simulink model "ASM_Traffic_MultiCore"  (R2026a)
settings: Solver=ode1  StartTime=SIM.tstart.v  StopTime=SIM.tend.v  FixedStep=SIM.StepSize.v
PostLoadFcn:
  | if any(exist('dsrtsu_mdlpostloadfcn', 'file') ~= 0), dsrtsu_mdlpostloadfcn('Execute', bdroot); end
  | try, asm_mdl_postloadfcn(bdroot, 'UpdateModel', 3600); catch, disp(lasterr); end,
InitFcn:
  | , if any(exist('rtifpga_mdlclblib', 'file') ~= 0), rtifpga_mdlclblib('Init', bdroot); end,
  | , if any(exist('dsmpb_private', 'file') ~= 0), dsmpb_private('dsmpb_mdlclblib', 'Init', bdroot); end,
model workspace (MAT data in the model file):
  asmReferencePath = [0 0.01 0.02 0.03 0.04 0.05 0.06 0.07 0.08 0.09 0.1 0.11 ... (350007 elements, 50001x7)]
  roadBounds : Simulink.Parameter (value not decoded)
  safetyAxes : Simulink.Parameter (value not decoded)
undefined symbols (not defined in the file): _to_, a0b2, ASM_BrakeHydraulics_DemoSystems, ASM_VehicleDynamics_DemoSystems, b98103fe8ad365046cd0, BrakeCircuit, controllerConfig, CPT, Crankshaft, DiscIntNeverNeededParam, dsmsi, FinalDriveAssembly, MDL, ModeSignals, mu, Pos_BrakePedal_Maneuver, rad, RefSignals, roadFamilyData, roadFamilyId, s_to_rpm, SIM, SoftECU, Suspension, Tire, Transmission
libraries: ASM_Traffic_lib x135, simulink x98, ASM_Utils_lib x77, ASM_VehicleDynamics_lib x70, ASM_Environment_lib x22, dsmpblib x20, dsmsilib x15, MDLD_Utils_lib x10, ASM_BrakeHydraulics_lib x3, sl_discontinuities x2
(part 63 of 65)

== system ASM_Traffic_MultiCore/VehicleDynamics/Plant/VehicleDynamics/VehicleMovement/ASMSignalCollector/Vehicle_Movement_Info_Car/Velocities ==
  CoGAndWheelVelocities : Inport
  v_Vehicle[x;y;z][m|s] : Inport  Port=2
  w_Vehicle[x;y;z][rad|s] : Inport  Port=3
  q_Wheel_dt[q1_Front;q2_Front;q1_Rear;q2_Rear][] : Inport  Port=4
  Bus Creator : BusCreator  Inputs=3
  Bus Selector : BusSelector  OutputSignals=v_Abs_Vehicle_CoG[x;y;z][km|h],w_CoG_VehicleBody[x;y;z][rad|s],WheelBodyVelocity,WheelBodyAngularVelocity,WheelAngularVelocity
  BusCreator1 : BusCreator  Inputs=2
  BusCreator2 : BusCreator  Inputs=2
  BusCreator4 : BusCreator  Inputs=3
  BusCreator5 : BusCreator  Inputs=1
  BusCreator6 : BusCreator  Inputs=1
  BusCreator7 : BusCreator  Inputs=2
  BusCreator8 : BusCreator  Inputs=3
  Selector : Selector  InputPortWidth=3  IndexOptions=Index vector (dialog)  Indices=[1 2]  OutputSizes=1
      settings: AttributesFormatString=Elements: %<Elements>
  VectorLabel : Subsystem
  VectorLabel3 : Subsystem
  VectorLabel4 : Subsystem
  "[m|s]_to_[km|h]" : Gain  Gain=3.6
  "[rad]_to_[deg]" : Gain  Gain=180/pi
  "[rad]_to_[deg]1" : Gain  Gain=180/pi
  v_Vehicle_and_AngleSideSlip : Subsystem
  Velocities : Outport  VectorParamsAs1DForOutWhenUnconnected=off
  wires:
  VectorLabel4/1(out) -> BusCreator8/3
  q_Wheel_dt[q1_Front;q2_Front;q1_Rear;q2_Rear][]/1 -> VectorLabel4/1(in)
  "[rad]_to_[deg]1"/1 -> BusCreator8/2  "w_Vehicle[x;y;z][deg|s]"
  "[rad]_to_[deg]"/1 -> VectorLabel3/1(in)
  w_Vehicle[x;y;z][rad|s]/1 -> "[rad]_to_[deg]1"/1
  BusCreator8/1 -> Bus Creator/3  "Generalized"
  v_Vehicle[x;y;z][m|s]/1 -> "[m|s]_to_[km|h]"/1
  "[m|s]_to_[km|h]"/1 -> BusCreator8/1  "v_Vehicle[x;y;z][km|h]"
  CoGAndWheelVelocities/1 -> Bus Selector/1
  BusCreator2/1 -> Bus Creator/1  "Vehicle"
  BusCreator4/1 -> BusCreator2/1  "Linear"
  BusCreator5/1 -> BusCreator2/2  "Angular"
  VectorLabel3/1(out) -> BusCreator5/1
  Bus Creator/1 -> Velocities/1  "Velocities"
  BusCreator1/1 -> Bus Creator/2  "Wheels"
  BusCreator7/1 -> BusCreator1/2  "Angular"
  Bus Selector/1 -> VectorLabel/1(in), Selector/1  "<v_Abs_Vehicle_CoG[x;y;z][km|h]>"
  BusCreator6/1 -> BusCreator1/1  "Linear"
  v_Vehicle_and_AngleSideSlip/1(v_Vehicle[km|h]) -> BusCreator4/2  "v_Total_Vehicle[km|h]"
  VectorLabel/1(out) -> BusCreator4/1
  Bus Selector/2 -> "[rad]_to_[deg]"/1  "<w_CoG_VehicleBody[x;y;z][rad|s]>"
  Bus Selector/3 -> BusCreator6/1  "<WheelBodyVelocity>"
  Bus Selector/4 -> BusCreator7/1  "<WheelBodyAngularVelocity>"
  Bus Selector/5 -> BusCreator7/2  "<WheelAngularVelocity>"
  Selector/1 -> v_Vehicle_and_AngleSideSlip/1(v_Vehicle[x;y][km|h])
  v_Vehicle_and_AngleSideSlip/2(Angle_SideSlip_Vehicle[deg]) -> BusCreator4/3  "Angle_SideSlip_Vehicle[deg]"

== system ASM_Traffic_MultiCore/DomainControl/DriverAssistance/Control/SoftECU_ACC/Soft_ECU_ACC/Map_Inputs/Maneuver/pos_edge_detection ==
  In1 : Inport
  Memory : Memory
  Relational Operator : RelationalOperator  Operator=>  OutDataTypeStr=boolean  InputSameDT=off
  Out1 : Outport  VectorParamsAs1DForOutWhenUnconnected=off
  wires:
  In1/1 -> Relational Operator/1, Memory/1
  Relational Operator/1 -> Out1/1
  Memory/1 -> Relational Operator/2

== system ASM_Traffic_MultiCore/DomainControl/DriverAssistance/Control/SoftECU_ACC/Soft_ECU_ACC/Map_Inputs/Maneuver/pos_edge_detection1 ==
  In1 : Inport
  Memory : Memory
  Relational Operator : RelationalOperator  Operator=>  OutDataTypeStr=boolean  InputSameDT=off
  Out1 : Outport  VectorParamsAs1DForOutWhenUnconnected=off
  wires:
  Memory/1 -> Relational Operator/2
  Relational Operator/1 -> Out1/1
  In1/1 -> Memory/1, Relational Operator/1

== system ASM_Traffic_MultiCore/DomainControl/DriverAssistance/Control/SoftECU_ACC/Soft_ECU_ACC/Map_Inputs/Maneuver/pos_edge_detection2 ==
  In1 : Inport
  Memory : Memory
  Relational Operator : RelationalOperator  Operator=>  OutDataTypeStr=boolean  InputSameDT=off
  Out1 : Outport  VectorParamsAs1DForOutWhenUnconnected=off
  wires:
  In1/1 -> Relational Operator/1, Memory/1
  Relational Operator/1 -> Out1/1
  Memory/1 -> Relational Operator/2

== system ASM_Traffic_MultiCore/DomainControl/DriverAssistance/Control/SoftECU_ACC/Soft_ECU_ACC/Map_Inputs/Maneuver/pos_edge_detection3 ==
  In1 : Inport
  Memory : Memory
  Relational Operator : RelationalOperator  Operator=>  OutDataTypeStr=boolean  InputSameDT=off
  Out1 : Outport  VectorParamsAs1DForOutWhenUnconnected=off
  wires:
  Memory/1 -> Relational Operator/2
  Relational Operator/1 -> Out1/1
  In1/1 -> Memory/1, Relational Operator/1

== system ASM_Traffic_MultiCore/Environment/GroundTruth/UserInterface/PAR_Plant/Fellow_Vehicles/Lightstates_Fellow1/Indicator_State[]/ASM_OSI_Mapping ==
  Fellow_TurnLights[] : Inport
  Table_ASM_To_OSI : Lookup_n-D  NumberOfTableDimensions=1  BreakpointsForDimension1=[0,1,2,3]  Table=[2,3,4,5]  InterpMethod=Nearest  InternalRulePriority=Speed  RndMeth=Simplest
  Indicator_State[] : Outport  VectorParamsAs1DForOutWhenUnconnected=off
  wires:
  Table_ASM_To_OSI/1 -> Indicator_State[]/1
  Fellow_TurnLights[]/1 -> Table_ASM_To_OSI/1

== system ASM_Traffic_MultiCore/Environment/GroundTruth/UserInterface/PAR_Plant/Fellow_Vehicles/Lightstates_Fellow10/Indicator_State[]/ASM_OSI_Mapping ==
  Fellow_TurnLights[] : Inport
  Table_ASM_To_OSI : Lookup_n-D  NumberOfTableDimensions=1  BreakpointsForDimension1=[0,1,2,3]  Table=[2,3,4,5]  InterpMethod=Nearest  InternalRulePriority=Speed  RndMeth=Simplest
  Indicator_State[] : Outport  VectorParamsAs1DForOutWhenUnconnected=off
  wires:
  Fellow_TurnLights[]/1 -> Table_ASM_To_OSI/1
  Table_ASM_To_OSI/1 -> Indicator_State[]/1

== system ASM_Traffic_MultiCore/Environment/GroundTruth/UserInterface/PAR_Plant/Fellow_Vehicles/Lightstates_Fellow11/Indicator_State[]/ASM_OSI_Mapping ==
  Fellow_TurnLights[] : Inport
  Table_ASM_To_OSI : Lookup_n-D  NumberOfTableDimensions=1  BreakpointsForDimension1=[0,1,2,3]  Table=[2,3,4,5]  InterpMethod=Nearest  InternalRulePriority=Speed  RndMeth=Simplest
  Indicator_State[] : Outport  VectorParamsAs1DForOutWhenUnconnected=off
  wires:
  Table_ASM_To_OSI/1 -> Indicator_State[]/1
  Fellow_TurnLights[]/1 -> Table_ASM_To_OSI/1

== system ASM_Traffic_MultiCore/Environment/GroundTruth/UserInterface/PAR_Plant/Fellow_Vehicles/Lightstates_Fellow12/Indicator_State[]/ASM_OSI_Mapping ==
  Fellow_TurnLights[] : Inport
  Table_ASM_To_OSI : Lookup_n-D  NumberOfTableDimensions=1  BreakpointsForDimension1=[0,1,2,3]  Table=[2,3,4,5]  InterpMethod=Nearest  InternalRulePriority=Speed  RndMeth=Simplest
  Indicator_State[] : Outport  VectorParamsAs1DForOutWhenUnconnected=off
  wires:
  Fellow_TurnLights[]/1 -> Table_ASM_To_OSI/1
  Table_ASM_To_OSI/1 -> Indicator_State[]/1

== system ASM_Traffic_MultiCore/Environment/GroundTruth/UserInterface/PAR_Plant/Fellow_Vehicles/Lightstates_Fellow13/Indicator_State[]/ASM_OSI_Mapping ==
  Fellow_TurnLights[] : Inport
  Table_ASM_To_OSI : Lookup_n-D  NumberOfTableDimensions=1  BreakpointsForDimension1=[0,1,2,3]  Table=[2,3,4,5]  InterpMethod=Nearest  InternalRulePriority=Speed  RndMeth=Simplest
  Indicator_State[] : Outport  VectorParamsAs1DForOutWhenUnconnected=off
  wires:
  Table_ASM_To_OSI/1 -> Indicator_State[]/1
  Fellow_TurnLights[]/1 -> Table_ASM_To_OSI/1

== system ASM_Traffic_MultiCore/Environment/GroundTruth/UserInterface/PAR_Plant/Fellow_Vehicles/Lightstates_Fellow14/Indicator_State[]/ASM_OSI_Mapping ==
  Fellow_TurnLights[] : Inport
  Table_ASM_To_OSI : Lookup_n-D  NumberOfTableDimensions=1  BreakpointsForDimension1=[0,1,2,3]  Table=[2,3,4,5]  InterpMethod=Nearest  InternalRulePriority=Speed  RndMeth=Simplest
  Indicator_State[] : Outport  VectorParamsAs1DForOutWhenUnconnected=off
  wires:
  Fellow_TurnLights[]/1 -> Table_ASM_To_OSI/1
  Table_ASM_To_OSI/1 -> Indicator_State[]/1

== system ASM_Traffic_MultiCore/Environment/GroundTruth/UserInterface/PAR_Plant/Fellow_Vehicles/Lightstates_Fellow15/Indicator_State[]/ASM_OSI_Mapping ==
  Fellow_TurnLights[] : Inport
  Table_ASM_To_OSI : Lookup_n-D  NumberOfTableDimensions=1  BreakpointsForDimension1=[0,1,2,3]  Table=[2,3,4,5]  InterpMethod=Nearest  InternalRulePriority=Speed  RndMeth=Simplest
  Indicator_State[] : Outport  VectorParamsAs1DForOutWhenUnconnected=off
  wires:
  Table_ASM_To_OSI/1 -> Indicator_State[]/1
  Fellow_TurnLights[]/1 -> Table_ASM_To_OSI/1

== system ASM_Traffic_MultiCore/Environment/GroundTruth/UserInterface/PAR_Plant/Fellow_Vehicles/Lightstates_Fellow16/Indicator_State[]/ASM_OSI_Mapping ==
  Fellow_TurnLights[] : Inport
  Table_ASM_To_OSI : Lookup_n-D  NumberOfTableDimensions=1  BreakpointsForDimension1=[0,1,2,3]  Table=[2,3,4,5]  InterpMethod=Nearest  InternalRulePriority=Speed  RndMeth=Simplest
  Indicator_State[] : Outport  VectorParamsAs1DForOutWhenUnconnected=off
  wires:
  Fellow_TurnLights[]/1 -> Table_ASM_To_OSI/1
  Table_ASM_To_OSI/1 -> Indicator_State[]/1

== system ASM_Traffic_MultiCore/Environment/GroundTruth/UserInterface/PAR_Plant/Fellow_Vehicles/Lightstates_Fellow17/Indicator_State[]/ASM_OSI_Mapping ==
  Fellow_TurnLights[] : Inport
  Table_ASM_To_OSI : Lookup_n-D  NumberOfTableDimensions=1  BreakpointsForDimension1=[0,1,2,3]  Table=[2,3,4,5]  InterpMethod=Nearest  InternalRulePriority=Speed  RndMeth=Simplest
  Indicator_State[] : Outport  VectorParamsAs1DForOutWhenUnconnected=off
  wires:
  Table_ASM_To_OSI/1 -> Indicator_State[]/1
  Fellow_TurnLights[]/1 -> Table_ASM_To_OSI/1

== system ASM_Traffic_MultiCore/Environment/GroundTruth/UserInterface/PAR_Plant/Fellow_Vehicles/Lightstates_Fellow18/Indicator_State[]/ASM_OSI_Mapping ==
  Fellow_TurnLights[] : Inport
  Table_ASM_To_OSI : Lookup_n-D  NumberOfTableDimensions=1  BreakpointsForDimension1=[0,1,2,3]  Table=[2,3,4,5]  InterpMethod=Nearest  InternalRulePriority=Speed  RndMeth=Simplest
  Indicator_State[] : Outport  VectorParamsAs1DForOutWhenUnconnected=off
  wires:
  Fellow_TurnLights[]/1 -> Table_ASM_To_OSI/1
  Table_ASM_To_OSI/1 -> Indicator_State[]/1

== system ASM_Traffic_MultiCore/Environment/GroundTruth/UserInterface/PAR_Plant/Fellow_Vehicles/Lightstates_Fellow19/Indicator_State[]/ASM_OSI_Mapping ==
  Fellow_TurnLights[] : Inport
  Table_ASM_To_OSI : Lookup_n-D  NumberOfTableDimensions=1  BreakpointsForDimension1=[0,1,2,3]  Table=[2,3,4,5]  InterpMethod=Nearest  InternalRulePriority=Speed  RndMeth=Simplest
  Indicator_State[] : Outport  VectorParamsAs1DForOutWhenUnconnected=off
  wires:
  Table_ASM_To_OSI/1 -> Indicator_State[]/1
  Fellow_TurnLights[]/1 -> Table_ASM_To_OSI/1

== system ASM_Traffic_MultiCore/Environment/GroundTruth/UserInterface/PAR_Plant/Fellow_Vehicles/Lightstates_Fellow2/Indicator_State[]/ASM_OSI_Mapping ==
  Fellow_TurnLights[] : Inport
  Table_ASM_To_OSI : Lookup_n-D  NumberOfTableDimensions=1  BreakpointsForDimension1=[0,1,2,3]  Table=[2,3,4,5]  InterpMethod=Nearest  InternalRulePriority=Speed  RndMeth=Simplest
  Indicator_State[] : Outport  VectorParamsAs1DForOutWhenUnconnected=off
  wires:
  Fellow_TurnLights[]/1 -> Table_ASM_To_OSI/1
  Table_ASM_To_OSI/1 -> Indicator_State[]/1

== system ASM_Traffic_MultiCore/Environment/GroundTruth/UserInterface/PAR_Plant/Fellow_Vehicles/Lightstates_Fellow20/Indicator_State[]/ASM_OSI_Mapping ==
  Fellow_TurnLights[] : Inport
  Table_ASM_To_OSI : Lookup_n-D  NumberOfTableDimensions=1  BreakpointsForDimension1=[0,1,2,3]  Table=[2,3,4,5]  InterpMethod=Nearest  InternalRulePriority=Speed  RndMeth=Simplest
  Indicator_State[] : Outport  VectorParamsAs1DForOutWhenUnconnected=off
  wires:
  Fellow_TurnLights[]/1 -> Table_ASM_To_OSI/1
  Table_ASM_To_OSI/1 -> Indicator_State[]/1

== system ASM_Traffic_MultiCore/Environment/GroundTruth/UserInterface/PAR_Plant/Fellow_Vehicles/Lightstates_Fellow21/Indicator_State[]/ASM_OSI_Mapping ==
  Fellow_TurnLights[] : Inport
  Table_ASM_To_OSI : Lookup_n-D  NumberOfTableDimensions=1  BreakpointsForDimension1=[0,1,2,3]  Table=[2,3,4,5]  InterpMethod=Nearest  InternalRulePriority=Speed  RndMeth=Simplest
  Indicator_State[] : Outport  VectorParamsAs1DForOutWhenUnconnected=off
  wires:
  Table_ASM_To_OSI/1 -> Indicator_State[]/1
  Fellow_TurnLights[]/1 -> Table_ASM_To_OSI/1

== system ASM_Traffic_MultiCore/Environment/GroundTruth/UserInterface/PAR_Plant/Fellow_Vehicles/Lightstates_Fellow22/Indicator_State[]/ASM_OSI_Mapping ==
  Fellow_TurnLights[] : Inport
  Table_ASM_To_OSI : Lookup_n-D  NumberOfTableDimensions=1  BreakpointsForDimension1=[0,1,2,3]  Table=[2,3,4,5]  InterpMethod=Nearest  InternalRulePriority=Speed  RndMeth=Simplest
  Indicator_State[] : Outport  VectorParamsAs1DForOutWhenUnconnected=off
  wires:
  Fellow_TurnLights[]/1 -> Table_ASM_To_OSI/1
  Table_ASM_To_OSI/1 -> Indicator_State[]/1

== system ASM_Traffic_MultiCore/Environment/GroundTruth/UserInterface/PAR_Plant/Fellow_Vehicles/Lightstates_Fellow23/Indicator_State[]/ASM_OSI_Mapping ==
  Fellow_TurnLights[] : Inport
  Table_ASM_To_OSI : Lookup_n-D  NumberOfTableDimensions=1  BreakpointsForDimension1=[0,1,2,3]  Table=[2,3,4,5]  InterpMethod=Nearest  InternalRulePriority=Speed  RndMeth=Simplest
  Indicator_State[] : Outport  VectorParamsAs1DForOutWhenUnconnected=off
  wires:
  Table_ASM_To_OSI/1 -> Indicator_State[]/1
  Fellow_TurnLights[]/1 -> Table_ASM_To_OSI/1

== system ASM_Traffic_MultiCore/Environment/GroundTruth/UserInterface/PAR_Plant/Fellow_Vehicles/Lightstates_Fellow24/Indicator_State[]/ASM_OSI_Mapping ==
  Fellow_TurnLights[] : Inport
  Table_ASM_To_OSI : Lookup_n-D  NumberOfTableDimensions=1  BreakpointsForDimension1=[0,1,2,3]  Table=[2,3,4,5]  InterpMethod=Nearest  InternalRulePriority=Speed  RndMeth=Simplest
  Indicator_State[] : Outport  VectorParamsAs1DForOutWhenUnconnected=off
  wires:
  Fellow_TurnLights[]/1 -> Table_ASM_To_OSI/1
  Table_ASM_To_OSI/1 -> Indicator_State[]/1

== system ASM_Traffic_MultiCore/Environment/GroundTruth/UserInterface/PAR_Plant/Fellow_Vehicles/Lightstates_Fellow25/Indicator_State[]/ASM_OSI_Mapping ==
  Fellow_TurnLights[] : Inport
  Table_ASM_To_OSI : Lookup_n-D  NumberOfTableDimensions=1  BreakpointsForDimension1=[0,1,2,3]  Table=[2,3,4,5]  InterpMethod=Nearest  InternalRulePriority=Speed  RndMeth=Simplest
  Indicator_State[] : Outport  VectorParamsAs1DForOutWhenUnconnected=off
  wires:
  Table_ASM_To_OSI/1 -> Indicator_State[]/1
  Fellow_TurnLights[]/1 -> Table_ASM_To_OSI/1

== system ASM_Traffic_MultiCore/Environment/GroundTruth/UserInterface/PAR_Plant/Fellow_Vehicles/Lightstates_Fellow26/Indicator_State[]/ASM_OSI_Mapping ==
  Fellow_TurnLights[] : Inport
  Table_ASM_To_OSI : Lookup_n-D  NumberOfTableDimensions=1  BreakpointsForDimension1=[0,1,2,3]  Table=[2,3,4,5]  InterpMethod=Nearest  InternalRulePriority=Speed  RndMeth=Simplest
  Indicator_State[] : Outport  VectorParamsAs1DForOutWhenUnconnected=off
  wires:
  Fellow_TurnLights[]/1 -> Table_ASM_To_OSI/1
  Table_ASM_To_OSI/1 -> Indicator_State[]/1

== system ASM_Traffic_MultiCore/Environment/GroundTruth/UserInterface/PAR_Plant/Fellow_Vehicles/Lightstates_Fellow27/Indicator_State[]/ASM_OSI_Mapping ==
  Fellow_TurnLights[] : Inport
  Table_ASM_To_OSI : Lookup_n-D  NumberOfTableDimensions=1  BreakpointsForDimension1=[0,1,2,3]  Table=[2,3,4,5]  InterpMethod=Nearest  InternalRulePriority=Speed  RndMeth=Simplest
  Indicator_State[] : Outport  VectorParamsAs1DForOutWhenUnconnected=off
  wires:
  Table_ASM_To_OSI/1 -> Indicator_State[]/1
  Fellow_TurnLights[]/1 -> Table_ASM_To_OSI/1

== system ASM_Traffic_MultiCore/Environment/GroundTruth/UserInterface/PAR_Plant/Fellow_Vehicles/Lightstates_Fellow28/Indicator_State[]/ASM_OSI_Mapping ==
  Fellow_TurnLights[] : Inport
  Table_ASM_To_OSI : Lookup_n-D  NumberOfTableDimensions=1  BreakpointsForDimension1=[0,1,2,3]  Table=[2,3,4,5]  InterpMethod=Nearest  InternalRulePriority=Speed  RndMeth=Simplest
  Indicator_State[] : Outport  VectorParamsAs1DForOutWhenUnconnected=off
  wires:
  Fellow_TurnLights[]/1 -> Table_ASM_To_OSI/1
  Table_ASM_To_OSI/1 -> Indicator_State[]/1

== system ASM_Traffic_MultiCore/Environment/GroundTruth/UserInterface/PAR_Plant/Fellow_Vehicles/Lightstates_Fellow29/Indicator_State[]/ASM_OSI_Mapping ==
  Fellow_TurnLights[] : Inport
  Table_ASM_To_OSI : Lookup_n-D  NumberOfTableDimensions=1  BreakpointsForDimension1=[0,1,2,3]  Table=[2,3,4,5]  InterpMethod=Nearest  InternalRulePriority=Speed  RndMeth=Simplest
  Indicator_State[] : Outport  VectorParamsAs1DForOutWhenUnconnected=off
  wires:
  Table_ASM_To_OSI/1 -> Indicator_State[]/1
  Fellow_TurnLights[]/1 -> Table_ASM_To_OSI/1

== system ASM_Traffic_MultiCore/Environment/GroundTruth/UserInterface/PAR_Plant/Fellow_Vehicles/Lightstates_Fellow3/Indicator_State[]/ASM_OSI_Mapping ==
  Fellow_TurnLights[] : Inport
  Table_ASM_To_OSI : Lookup_n-D  NumberOfTableDimensions=1  BreakpointsForDimension1=[0,1,2,3]  Table=[2,3,4,5]  InterpMethod=Nearest  InternalRulePriority=Speed  RndMeth=Simplest
  Indicator_State[] : Outport  VectorParamsAs1DForOutWhenUnconnected=off
  wires:
  Table_ASM_To_OSI/1 -> Indicator_State[]/1
  Fellow_TurnLights[]/1 -> Table_ASM_To_OSI/1

== system ASM_Traffic_MultiCore/Environment/GroundTruth/UserInterface/PAR_Plant/Fellow_Vehicles/Lightstates_Fellow30/Indicator_State[]/ASM_OSI_Mapping ==
  Fellow_TurnLights[] : Inport
  Table_ASM_To_OSI : Lookup_n-D  NumberOfTableDimensions=1  BreakpointsForDimension1=[0,1,2,3]  Table=[2,3,4,5]  InterpMethod=Nearest  InternalRulePriority=Speed  RndMeth=Simplest
  Indicator_State[] : Outport  VectorParamsAs1DForOutWhenUnconnected=off
  wires:
  Fellow_TurnLights[]/1 -> Table_ASM_To_OSI/1
  Table_ASM_To_OSI/1 -> Indicator_State[]/1

== system ASM_Traffic_MultiCore/Environment/GroundTruth/UserInterface/PAR_Plant/Fellow_Vehicles/Lightstates_Fellow4/Indicator_State[]/ASM_OSI_Mapping ==
  Fellow_TurnLights[] : Inport
  Table_ASM_To_OSI : Lookup_n-D  NumberOfTableDimensions=1  BreakpointsForDimension1=[0,1,2,3]  Table=[2,3,4,5]  InterpMethod=Nearest  InternalRulePriority=Speed  RndMeth=Simplest
  Indicator_State[] : Outport  VectorParamsAs1DForOutWhenUnconnected=off
  wires:
  Fellow_TurnLights[]/1 -> Table_ASM_To_OSI/1
  Table_ASM_To_OSI/1 -> Indicator_State[]/1

== system ASM_Traffic_MultiCore/Environment/GroundTruth/UserInterface/PAR_Plant/Fellow_Vehicles/Lightstates_Fellow5/Indicator_State[]/ASM_OSI_Mapping ==
  Fellow_TurnLights[] : Inport
  Table_ASM_To_OSI : Lookup_n-D  NumberOfTableDimensions=1  BreakpointsForDimension1=[0,1,2,3]  Table=[2,3,4,5]  InterpMethod=Nearest  InternalRulePriority=Speed  RndMeth=Simplest
  Indicator_State[] : Outport  VectorParamsAs1DForOutWhenUnconnected=off
  wires:
  Table_ASM_To_OSI/1 -> Indicator_State[]/1
  Fellow_TurnLights[]/1 -> Table_ASM_To_OSI/1

== system ASM_Traffic_MultiCore/Environment/GroundTruth/UserInterface/PAR_Plant/Fellow_Vehicles/Lightstates_Fellow6/Indicator_State[]/ASM_OSI_Mapping ==
  Fellow_TurnLights[] : Inport
  Table_ASM_To_OSI : Lookup_n-D  NumberOfTableDimensions=1  BreakpointsForDimension1=[0,1,2,3]  Table=[2,3,4,5]  InterpMethod=Nearest  InternalRulePriority=Speed  RndMeth=Simplest
  Indicator_State[] : Outport  VectorParamsAs1DForOutWhenUnconnected=off
  wires:
  Fellow_TurnLights[]/1 -> Table_ASM_To_OSI/1
  Table_ASM_To_OSI/1 -> Indicator_State[]/1

== system ASM_Traffic_MultiCore/Environment/GroundTruth/UserInterface/PAR_Plant/Fellow_Vehicles/Lightstates_Fellow7/Indicator_State[]/ASM_OSI_Mapping ==
  Fellow_TurnLights[] : Inport
  Table_ASM_To_OSI : Lookup_n-D  NumberOfTableDimensions=1  BreakpointsForDimension1=[0,1,2,3]  Table=[2,3,4,5]  InterpMethod=Nearest  InternalRulePriority=Speed  RndMeth=Simplest
  Indicator_State[] : Outport  VectorParamsAs1DForOutWhenUnconnected=off
  wires:
  Table_ASM_To_OSI/1 -> Indicator_State[]/1
  Fellow_TurnLights[]/1 -> Table_ASM_To_OSI/1

== system ASM_Traffic_MultiCore/Environment/GroundTruth/UserInterface/PAR_Plant/Fellow_Vehicles/Lightstates_Fellow8/Indicator_State[]/ASM_OSI_Mapping ==
  Fellow_TurnLights[] : Inport
  Table_ASM_To_OSI : Lookup_n-D  NumberOfTableDimensions=1  BreakpointsForDimension1=[0,1,2,3]  Table=[2,3,4,5]  InterpMethod=Nearest  InternalRulePriority=Speed  RndMeth=Simplest
  Indicator_State[] : Outport  VectorParamsAs1DForOutWhenUnconnected=off
  wires:
  Fellow_TurnLights[]/1 -> Table_ASM_To_OSI/1
  Table_ASM_To_OSI/1 -> Indicator_State[]/1

== system ASM_Traffic_MultiCore/Environment/GroundTruth/UserInterface/PAR_Plant/Fellow_Vehicles/Lightstates_Fellow9/Indicator_State[]/ASM_OSI_Mapping ==
  Fellow_TurnLights[] : Inport
  Table_ASM_To_OSI : Lookup_n-D  NumberOfTableDimensions=1  BreakpointsForDimension1=[0,1,2,3]  Table=[2,3,4,5]  InterpMethod=Nearest  InternalRulePriority=Speed  RndMeth=Simplest
  Indicator_State[] : Outport  VectorParamsAs1DForOutWhenUnconnected=off
  wires:
  Table_ASM_To_OSI/1 -> Indicator_State[]/1
  Fellow_TurnLights[]/1 -> Table_ASM_To_OSI/1

== system ASM_Traffic_MultiCore/Environment/Sensors/PlantModel/Object_Sensor_2D/ObjectData/Sensor1/Object_Custom_Values/Vectorize_Signals ==
  SensorOutput1 : Inport
  SensorOutput2 : Inport  Port=2
  SensorOutput3 : Inport  Port=3
  Bus Creator : BusCreator  Inputs=2
  Bus Selector : BusSelector  OutputSignals=SensorOutput.Object1.Object_Valid[0|1],SensorOutput.Object2.Object_Valid[0|1],SensorOutput.Object3.Object_Valid[0|1],SensorOutput.Object4.Object_Valid[0|1],SensorOutput.Object5.Object_Valid[0|1]
  Bus Selector1 : BusSelector  OutputSignals=SensorOutput.Object1.Object_Valid[0|1],SensorOutput.Object2.Object_Valid[0|1],SensorOutput.Object3.Object_Valid[0|1],SensorOutput.Object4.Object_Valid[0|1],SensorOutput.Object5.Object_Valid[0|1]
  Bus Selector2 : BusSelector  OutputSignals=SensorOutput.Object1.Object_Valid[0|1],SensorOutput.Object2.Object_Valid[0|1],SensorOutput.Object3.Object_Valid[0|1],SensorOutput.Object4.Object_Valid[0|1],SensorOutput.Object5.Object_Valid[0|1]
  Bus Selector3 : BusSelector  OutputSignals=SensorOutput.Object1.CustomValues[],SensorOutput.Object2.CustomValues[],SensorOutput.Object3.CustomValues[],SensorOutput.Object4.CustomValues[],SensorOutput.Object5.CustomValues[]
  Bus Selector4 : BusSelector  OutputSignals=SensorOutput.Object1.CustomValues[],SensorOutput.Object2.CustomValues[],SensorOutput.Object3.CustomValues[],SensorOutput.Object4.CustomValues[],SensorOutput.Object5.CustomValues[]
  Bus Selector5 : BusSelector  OutputSignals=SensorOutput.Object1.CustomValues[],SensorOutput.Object2.CustomValues[],SensorOutput.Object3.CustomValues[],SensorOutput.Object4.CustomValues[],SensorOutput.Object5.CustomValues[]
  Mux : Mux  Inputs=15
  Mux1 : Mux  Inputs=15
  Vectorized_Custom_Values : Outport  VectorParamsAs1DForOutWhenUnconnected=off
  wires:
  Bus Creator/1 -> Vectorized_Custom_Values/1
  Bus Selector5/5 -> Mux1/15  "<CustomValues[]>"
  Bus Selector5/4 -> Mux1/14  "<CustomValues[]>"
  Bus Selector5/3 -> Mux1/13  "<CustomValues[]>"
  Bus Selector5/2 -> Mux1/12  "<CustomValues[]>"
  Bus Selector5/1 -> Mux1/11  "<CustomValues[]>"
  Bus Selector4/5 -> Mux1/10  "<CustomValues[]>"
  Bus Selector4/4 -> Mux1/9  "<CustomValues[]>"
  Bus Selector4/3 -> Mux1/8  "<CustomValues[]>"
  Bus Selector4/2 -> Mux1/7  "<CustomValues[]>"
  Bus Selector4/1 -> Mux1/6  "<CustomValues[]>"
  Bus Selector3/5 -> Mux1/5  "<CustomValues[]>"
  Bus Selector3/4 -> Mux1/4  "<CustomValues[]>"
  Bus Selector3/3 -> Mux1/3  "<CustomValues[]>"
  Bus Selector3/2 -> Mux1/2  "<CustomValues[]>"
  Bus Selector3/1 -> Mux1/1  "<CustomValues[]>"
  Bus Selector2/5 -> Mux/15  "<Object_Valid[0|1]>"
  Bus Selector2/4 -> Mux/14  "<Object_Valid[0|1]>"
  Bus Selector2/3 -> Mux/13  "<Object_Valid[0|1]>"
  Bus Selector2/2 -> Mux/12  "<Object_Valid[0|1]>"
  Bus Selector2/1 -> Mux/11  "<Object_Valid[0|1]>"
  Bus Selector1/5 -> Mux/10  "<Object_Valid[0|1]>"
  Bus Selector1/4 -> Mux/9  "<Object_Valid[0|1]>"
  Bus Selector1/3 -> Mux/8  "<Object_Valid[0|1]>"
  Bus Selector1/2 -> Mux/7  "<Object_Valid[0|1]>"
  Bus Selector1/1 -> Mux/6  "<Object_Valid[0|1]>"
  Mux1/1 -> Bus Creator/2  "CustomValues[]"
  Mux/1 -> Bus Creator/1  "Object_Valid[0|1]"
  SensorOutput3/1 -> Bus Selector2/1, Bus Selector5/1
  SensorOutput2/1 -> Bus Selector1/1, Bus Selector4/1
  Bus Selector/1 -> Mux/1  "<Object_Valid[0|1]>"
  Bus Selector/2 -> Mux/2  "<Object_Valid[0|1]>"
  Bus Selector/3 -> Mux/3  "<Object_Valid[0|1]>"
  Bus Selector/4 -> Mux/4  "<Object_Valid[0|1]>"
  Bus Selector/5 -> Mux/5  "<Object_Valid[0|1]>"
  SensorOutput1/1 -> Bus Selector3/1, Bus Selector/1

== system ASM_Traffic_MultiCore/Environment/Sensors/PlantModel/Object_Sensor_2D/ObjectData/Sensor2/Object_Custom_Values/Vectorize_Signals ==
  SensorOutput1 : Inport
  SensorOutput2 : Inport  Port=2
  SensorOutput3 : Inport  Port=3
  Bus Creator : BusCreator  Inputs=2
  Bus Selector : BusSelector  OutputSignals=SensorOutput.Object1.Object_Valid[0|1],SensorOutput.Object2.Object_Valid[0|1],SensorOutput.Object3.Object_Valid[0|1],SensorOutput.Object4.Object_Valid[0|1],SensorOutput.Object5.Object_Valid[0|1]
  Bus Selector1 : BusSelector  OutputSignals=SensorOutput.Object1.Object_Valid[0|1],SensorOutput.Object2.Object_Valid[0|1],SensorOutput.Object3.Object_Valid[0|1],SensorOutput.Object4.Object_Valid[0|1],SensorOutput.Object5.Object_Valid[0|1]
  Bus Selector2 : BusSelector  OutputSignals=SensorOutput.Object1.Object_Valid[0|1],SensorOutput.Object2.Object_Valid[0|1],SensorOutput.Object3.Object_Valid[0|1],SensorOutput.Object4.Object_Valid[0|1],SensorOutput.Object5.Object_Valid[0|1]
  Bus Selector3 : BusSelector  OutputSignals=SensorOutput.Object1.CustomValues[],SensorOutput.Object2.CustomValues[],SensorOutput.Object3.CustomValues[],SensorOutput.Object4.CustomValues[],SensorOutput.Object5.CustomValues[]
  Bus Selector4 : BusSelector  OutputSignals=SensorOutput.Object1.CustomValues[],SensorOutput.Object2.CustomValues[],SensorOutput.Object3.CustomValues[],SensorOutput.Object4.CustomValues[],SensorOutput.Object5.CustomValues[]
  Bus Selector5 : BusSelector  OutputSignals=SensorOutput.Object1.CustomValues[],SensorOutput.Object2.CustomValues[],SensorOutput.Object3.CustomValues[],SensorOutput.Object4.CustomValues[],SensorOutput.Object5.CustomValues[]
  Mux : Mux  Inputs=15
  Mux1 : Mux  Inputs=15
  Vectorized_Custom_Values : Outport  VectorParamsAs1DForOutWhenUnconnected=off
  wires:
  SensorOutput1/1 -> Bus Selector/1, Bus Selector3/1
  Bus Selector/5 -> Mux/5  "<Object_Valid[0|1]>"
  Bus Selector/4 -> Mux/4  "<Object_Valid[0|1]>"
  Bus Selector/3 -> Mux/3  "<Object_Valid[0|1]>"
  Bus Selector/2 -> Mux/2  "<Object_Valid[0|1]>"
  Bus Selector/1 -> Mux/1  "<Object_Valid[0|1]>"
  SensorOutput2/1 -> Bus Selector4/1, Bus Selector1/1
  SensorOutput3/1 -> Bus Selector5/1, Bus Selector2/1
  Mux/1 -> Bus Creator/1  "Object_Valid[0|1]"
  Mux1/1 -> Bus Creator/2  "CustomValues[]"
  Bus Selector1/1 -> Mux/6  "<Object_Valid[0|1]>"
  Bus Selector1/2 -> Mux/7  "<Object_Valid[0|1]>"
  Bus Selector1/3 -> Mux/8  "<Object_Valid[0|1]>"
  Bus Selector1/4 -> Mux/9  "<Object_Valid[0|1]>"
  Bus Selector1/5 -> Mux/10  "<Object_Valid[0|1]>"
  Bus Selector2/1 -> Mux/11  "<Object_Valid[0|1]>"
  Bus Selector2/2 -> Mux/12  "<Object_Valid[0|1]>"
  Bus Selector2/3 -> Mux/13  "<Object_Valid[0|1]>"
  Bus Selector2/4 -> Mux/14  "<Object_Valid[0|1]>"
  Bus Selector2/5 -> Mux/15  "<Object_Valid[0|1]>"
  Bus Selector3/1 -> Mux1/1  "<CustomValues[]>"
  Bus Selector3/2 -> Mux1/2  "<CustomValues[]>"
  Bus Selector3/3 -> Mux1/3  "<CustomValues[]>"
  Bus Selector3/4 -> Mux1/4  "<CustomValues[]>"
  Bus Selector3/5 -> Mux1/5  "<CustomValues[]>"
  Bus Selector4/1 -> Mux1/6  "<CustomValues[]>"
  Bus Selector4/2 -> Mux1/7  "<CustomValues[]>"
  Bus Selector4/3 -> Mux1/8  "<CustomValues[]>"
  Bus Selector4/4 -> Mux1/9  "<CustomValues[]>"
  Bus Selector4/5 -> Mux1/10  "<CustomValues[]>"
  Bus Selector5/1 -> Mux1/11  "<CustomValues[]>"
  Bus Selector5/2 -> Mux1/12  "<CustomValues[]>"
  Bus Selector5/3 -> Mux1/13  "<CustomValues[]>"
  Bus Selector5/4 -> Mux1/14  "<CustomValues[]>"
  Bus Selector5/5 -> Mux1/15  "<CustomValues[]>"
  Bus Creator/1 -> Vectorized_Custom_Values/1

== system ASM_Traffic_MultiCore/Environment/Sensors/PlantModel/Object_Sensor_2D/ObjectData/Sensor3/Object_Custom_Values/Vectorize_Signals ==
  SensorOutput1 : Inport
  SensorOutput2 : Inport  Port=2
  SensorOutput3 : Inport  Port=3
  Bus Creator : BusCreator  Inputs=2
  Bus Selector : BusSelector  OutputSignals=SensorOutput.Object1.Object_Valid[0|1],SensorOutput.Object2.Object_Valid[0|1],SensorOutput.Object3.Object_Valid[0|1],SensorOutput.Object4.Object_Valid[0|1],SensorOutput.Object5.Object_Valid[0|1]
  Bus Selector1 : BusSelector  OutputSignals=SensorOutput.Object1.Object_Valid[0|1],SensorOutput.Object2.Object_Valid[0|1],SensorOutput.Object3.Object_Valid[0|1],SensorOutput.Object4.Object_Valid[0|1],SensorOutput.Object5.Object_Valid[0|1]
  Bus Selector2 : BusSelector  OutputSignals=SensorOutput.Object1.Object_Valid[0|1],SensorOutput.Object2.Object_Valid[0|1],SensorOutput.Object3.Object_Valid[0|1],SensorOutput.Object4.Object_Valid[0|1],SensorOutput.Object5.Object_Valid[0|1]
  Bus Selector3 : BusSelector  OutputSignals=SensorOutput.Object1.CustomValues[],SensorOutput.Object2.CustomValues[],SensorOutput.Object3.CustomValues[],SensorOutput.Object4.CustomValues[],SensorOutput.Object5.CustomValues[]
  Bus Selector4 : BusSelector  OutputSignals=SensorOutput.Object1.CustomValues[],SensorOutput.Object2.CustomValues[],SensorOutput.Object3.CustomValues[],SensorOutput.Object4.CustomValues[],SensorOutput.Object5.CustomValues[]
  Bus Selector5 : BusSelector  OutputSignals=SensorOutput.Object1.CustomValues[],SensorOutput.Object2.CustomValues[],SensorOutput.Object3.CustomValues[],SensorOutput.Object4.CustomValues[],SensorOutput.Object5.CustomValues[]
  Mux : Mux  Inputs=15
  Mux1 : Mux  Inputs=15
  Vectorized_Custom_Values : Outport  VectorParamsAs1DForOutWhenUnconnected=off
  wires:
  Bus Creator/1 -> Vectorized_Custom_Values/1
  Bus Selector5/5 -> Mux1/15  "<CustomValues[]>"
  Bus Selector5/4 -> Mux1/14  "<CustomValues[]>"
  Bus Selector5/3 -> Mux1/13  "<CustomValues[]>"
  Bus Selector5/2 -> Mux1/12  "<CustomValues[]>"
  Bus Selector5/1 -> Mux1/11  "<CustomValues[]>"
  Bus Selector4/5 -> Mux1/10  "<CustomValues[]>"
  Bus Selector4/4 -> Mux1/9  "<CustomValues[]>"
  Bus Selector4/3 -> Mux1/8  "<CustomValues[]>"
  Bus Selector4/2 -> Mux1/7  "<CustomValues[]>"
  Bus Selector4/1 -> Mux1/6  "<CustomValues[]>"
  Bus Selector3/5 -> Mux1/5  "<CustomValues[]>"
  Bus Selector3/4 -> Mux1/4  "<CustomValues[]>"
  Bus Selector3/3 -> Mux1/3  "<CustomValues[]>"
  Bus Selector3/2 -> Mux1/2  "<CustomValues[]>"
  Bus Selector3/1 -> Mux1/1  "<CustomValues[]>"
  Bus Selector2/5 -> Mux/15  "<Object_Valid[0|1]>"
  Bus Selector2/4 -> Mux/14  "<Object_Valid[0|1]>"
  Bus Selector2/3 -> Mux/13  "<Object_Valid[0|1]>"
  Bus Selector2/2 -> Mux/12  "<Object_Valid[0|1]>"
  Bus Selector2/1 -> Mux/11  "<Object_Valid[0|1]>"
  Bus Selector1/5 -> Mux/10  "<Object_Valid[0|1]>"
  Bus Selector1/4 -> Mux/9  "<Object_Valid[0|1]>"
  Bus Selector1/3 -> Mux/8  "<Object_Valid[0|1]>"
  Bus Selector1/2 -> Mux/7  "<Object_Valid[0|1]>"
  Bus Selector1/1 -> Mux/6  "<Object_Valid[0|1]>"
  Mux1/1 -> Bus Creator/2  "CustomValues[]"
  Mux/1 -> Bus Creator/1  "Object_Valid[0|1]"
  SensorOutput3/1 -> Bus Selector2/1, Bus Selector5/1
  SensorOutput2/1 -> Bus Selector1/1, Bus Selector4/1
  Bus Selector/1 -> Mux/1  "<Object_Valid[0|1]>"
  Bus Selector/2 -> Mux/2  "<Object_Valid[0|1]>"
  Bus Selector/3 -> Mux/3  "<Object_Valid[0|1]>"
  Bus Selector/4 -> Mux/4  "<Object_Valid[0|1]>"
  Bus Selector/5 -> Mux/5  "<Object_Valid[0|1]>"
  SensorOutput1/1 -> Bus Selector3/1, Bus Selector/1

== system ASM_Traffic_MultiCore/Environment/Sensors/PlantModel/Object_Sensor_2D/ObjectData/Sensor4/Object_Custom_Values/Vectorize_Signals ==
  SensorOutput1 : Inport
  SensorOutput2 : Inport  Port=2
  SensorOutput3 : Inport  Port=3
  Bus Creator : BusCreator  Inputs=2
  Bus Selector : BusSelector  OutputSignals=SensorOutput.Object1.Object_Valid[0|1],SensorOutput.Object2.Object_Valid[0|1],SensorOutput.Object3.Object_Valid[0|1],SensorOutput.Object4.Object_Valid[0|1],SensorOutput.Object5.Object_Valid[0|1]
  Bus Selector1 : BusSelector  OutputSignals=SensorOutput.Object1.Object_Valid[0|1],SensorOutput.Object2.Object_Valid[0|1],SensorOutput.Object3.Object_Valid[0|1],SensorOutput.Object4.Object_Valid[0|1],SensorOutput.Object5.Object_Valid[0|1]
  Bus Selector2 : BusSelector  OutputSignals=SensorOutput.Object1.Object_Valid[0|1],SensorOutput.Object2.Object_Valid[0|1],SensorOutput.Object3.Object_Valid[0|1],SensorOutput.Object4.Object_Valid[0|1],SensorOutput.Object5.Object_Valid[0|1]
  Bus Selector3 : BusSelector  OutputSignals=SensorOutput.Object1.CustomValues[],SensorOutput.Object2.CustomValues[],SensorOutput.Object3.CustomValues[],SensorOutput.Object4.CustomValues[],SensorOutput.Object5.CustomValues[]
  Bus Selector4 : BusSelector  OutputSignals=SensorOutput.Object1.CustomValues[],SensorOutput.Object2.CustomValues[],SensorOutput.Object3.CustomValues[],SensorOutput.Object4.CustomValues[],SensorOutput.Object5.CustomValues[]
  Bus Selector5 : BusSelector  OutputSignals=SensorOutput.Object1.CustomValues[],SensorOutput.Object2.CustomValues[],SensorOutput.Object3.CustomValues[],SensorOutput.Object4.CustomValues[],SensorOutput.Object5.CustomValues[]
  Mux : Mux  Inputs=15
  Mux1 : Mux  Inputs=15
  Vectorized_Custom_Values : Outport  VectorParamsAs1DForOutWhenUnconnected=off
  wires:
  Bus Creator/1 -> Vectorized_Custom_Values/1
  Bus Selector5/5 -> Mux1/15  "<CustomValues[]>"
  Bus Selector5/4 -> Mux1/14  "<CustomValues[]>"
  Bus Selector5/3 -> Mux1/13  "<CustomValues[]>"
  Bus Selector5/2 -> Mux1/12  "<CustomValues[]>"
  Bus Selector5/1 -> Mux1/11  "<CustomValues[]>"
  Bus Selector4/5 -> Mux1/10  "<CustomValues[]>"
  Bus Selector4/4 -> Mux1/9  "<CustomValues[]>"
  Bus Selector4/3 -> Mux1/8  "<CustomValues[]>"
  Bus Selector4/2 -> Mux1/7  "<CustomValues[]>"
  Bus Selector4/1 -> Mux1/6  "<CustomValues[]>"
  Bus Selector3/5 -> Mux1/5  "<CustomValues[]>"
  Bus Selector3/4 -> Mux1/4  "<CustomValues[]>"
  Bus Selector3/3 -> Mux1/3  "<CustomValues[]>"
  Bus Selector3/2 -> Mux1/2  "<CustomValues[]>"
  Bus Selector3/1 -> Mux1/1  "<CustomValues[]>"
  Bus Selector2/5 -> Mux/15  "<Object_Valid[0|1]>"
  Bus Selector2/4 -> Mux/14  "<Object_Valid[0|1]>"
  Bus Selector2/3 -> Mux/13  "<Object_Valid[0|1]>"
  Bus Selector2/2 -> Mux/12  "<Object_Valid[0|1]>"
  Bus Selector2/1 -> Mux/11  "<Object_Valid[0|1]>"
  Bus Selector1/5 -> Mux/10  "<Object_Valid[0|1]>"
  Bus Selector1/4 -> Mux/9  "<Object_Valid[0|1]>"
  Bus Selector1/3 -> Mux/8  "<Object_Valid[0|1]>"
  Bus Selector1/2 -> Mux/7  "<Object_Valid[0|1]>"
  Bus Selector1/1 -> Mux/6  "<Object_Valid[0|1]>"
  Mux1/1 -> Bus Creator/2  "CustomValues[]"
  Mux/1 -> Bus Creator/1  "Object_Valid[0|1]"
  SensorOutput3/1 -> Bus Selector2/1, Bus Selector5/1
  SensorOutput2/1 -> Bus Selector1/1, Bus Selector4/1
  Bus Selector/1 -> Mux/1  "<Object_Valid[0|1]>"
  Bus Selector/2 -> Mux/2  "<Object_Valid[0|1]>"
  Bus Selector/3 -> Mux/3  "<Object_Valid[0|1]>"
  Bus Selector/4 -> Mux/4  "<Object_Valid[0|1]>"
  Bus Selector/5 -> Mux/5  "<Object_Valid[0|1]>"
  SensorOutput1/1 -> Bus Selector3/1, Bus Selector/1

== system ASM_Traffic_MultiCore/Environment/Sensors/PlantModel/Object_Sensor_2D/ObjectData/Sensor5/Object_Custom_Values/Vectorize_Signals ==
  SensorOutput1 : Inport
  SensorOutput2 : Inport  Port=2
  SensorOutput3 : Inport  Port=3
  Bus Creator : BusCreator  Inputs=2
  Bus Selector : BusSelector  OutputSignals=SensorOutput.Object1.Object_Valid[0|1],SensorOutput.Object2.Object_Valid[0|1],SensorOutput.Object3.Object_Valid[0|1],SensorOutput.Object4.Object_Valid[0|1],SensorOutput.Object5.Object_Valid[0|1]
  Bus Selector1 : BusSelector  OutputSignals=SensorOutput.Object1.Object_Valid[0|1],SensorOutput.Object2.Object_Valid[0|1],SensorOutput.Object3.Object_Valid[0|1],SensorOutput.Object4.Object_Valid[0|1],SensorOutput.Object5.Object_Valid[0|1]
  Bus Selector2 : BusSelector  OutputSignals=SensorOutput.Object1.Object_Valid[0|1],SensorOutput.Object2.Object_Valid[0|1],SensorOutput.Object3.Object_Valid[0|1],SensorOutput.Object4.Object_Valid[0|1],SensorOutput.Object5.Object_Valid[0|1]
  Bus Selector3 : BusSelector  OutputSignals=SensorOutput.Object1.CustomValues[],SensorOutput.Object2.CustomValues[],SensorOutput.Object3.CustomValues[],SensorOutput.Object4.CustomValues[],SensorOutput.Object5.CustomValues[]
  Bus Selector4 : BusSelector  OutputSignals=SensorOutput.Object1.CustomValues[],SensorOutput.Object2.CustomValues[],SensorOutput.Object3.CustomValues[],SensorOutput.Object4.CustomValues[],SensorOutput.Object5.CustomValues[]
  Bus Selector5 : BusSelector  OutputSignals=SensorOutput.Object1.CustomValues[],SensorOutput.Object2.CustomValues[],SensorOutput.Object3.CustomValues[],SensorOutput.Object4.CustomValues[],SensorOutput.Object5.CustomValues[]
  Mux : Mux  Inputs=15
  Mux1 : Mux  Inputs=15
  Vectorized_Custom_Values : Outport  VectorParamsAs1DForOutWhenUnconnected=off
  wires:
  SensorOutput1/1 -> Bus Selector/1, Bus Selector3/1
  Bus Selector/5 -> Mux/5  "<Object_Valid[0|1]>"
  Bus Selector/4 -> Mux/4  "<Object_Valid[0|1]>"
  Bus Selector/3 -> Mux/3  "<Object_Valid[0|1]>"
  Bus Selector/2 -> Mux/2  "<Object_Valid[0|1]>"
  Bus Selector/1 -> Mux/1  "<Object_Valid[0|1]>"
  SensorOutput2/1 -> Bus Selector4/1, Bus Selector1/1
  SensorOutput3/1 -> Bus Selector5/1, Bus Selector2/1
  Mux/1 -> Bus Creator/1  "Object_Valid[0|1]"
  Mux1/1 -> Bus Creator/2  "CustomValues[]"
  Bus Selector1/1 -> Mux/6  "<Object_Valid[0|1]>"
  Bus Selector1/2 -> Mux/7  "<Object_Valid[0|1]>"
  Bus Selector1/3 -> Mux/8  "<Object_Valid[0|1]>"
  Bus Selector1/4 -> Mux/9  "<Object_Valid[0|1]>"
  Bus Selector1/5 -> Mux/10  "<Object_Valid[0|1]>"
  Bus Selector2/1 -> Mux/11  "<Object_Valid[0|1]>"
  Bus Selector2/2 -> Mux/12  "<Object_Valid[0|1]>"
  Bus Selector2/3 -> Mux/13  "<Object_Valid[0|1]>"
  Bus Selector2/4 -> Mux/14  "<Object_Valid[0|1]>"
  Bus Selector2/5 -> Mux/15  "<Object_Valid[0|1]>"
  Bus Selector3/1 -> Mux1/1  "<CustomValues[]>"
  Bus Selector3/2 -> Mux1/2  "<CustomValues[]>"
  Bus Selector3/3 -> Mux1/3  "<CustomValues[]>"
  Bus Selector3/4 -> Mux1/4  "<CustomValues[]>"
  Bus Selector3/5 -> Mux1/5  "<CustomValues[]>"
  Bus Selector4/1 -> Mux1/6  "<CustomValues[]>"
  Bus Selector4/2 -> Mux1/7  "<CustomValues[]>"
  Bus Selector4/3 -> Mux1/8  "<CustomValues[]>"
  Bus Selector4/4 -> Mux1/9  "<CustomValues[]>"
  Bus Selector4/5 -> Mux1/10  "<CustomValues[]>"
  Bus Selector5/1 -> Mux1/11  "<CustomValues[]>"
  Bus Selector5/2 -> Mux1/12  "<CustomValues[]>"
  Bus Selector5/3 -> Mux1/13  "<CustomValues[]>"
  Bus Selector5/4 -> Mux1/14  "<CustomValues[]>"
  Bus Selector5/5 -> Mux1/15  "<CustomValues[]>"
  Bus Creator/1 -> Vectorized_Custom_Values/1

== system ASM_Traffic_MultiCore/Environment/Sensors/PlantModel/Object_Sensor_2D/ObjectData/Sensor6/Object_Custom_Values/Vectorize_Signals ==
  SensorOutput1 : Inport
  SensorOutput2 : Inport  Port=2
  SensorOutput3 : Inport  Port=3
  Bus Creator : BusCreator  Inputs=2
  Bus Selector : BusSelector  OutputSignals=SensorOutput.Object1.Object_Valid[0|1],SensorOutput.Object2.Object_Valid[0|1],SensorOutput.Object3.Object_Valid[0|1],SensorOutput.Object4.Object_Valid[0|1],SensorOutput.Object5.Object_Valid[0|1]
  Bus Selector1 : BusSelector  OutputSignals=SensorOutput.Object1.Object_Valid[0|1],SensorOutput.Object2.Object_Valid[0|1],SensorOutput.Object3.Object_Valid[0|1],SensorOutput.Object4.Object_Valid[0|1],SensorOutput.Object5.Object_Valid[0|1]
  Bus Selector2 : BusSelector  OutputSignals=SensorOutput.Object1.Object_Valid[0|1],SensorOutput.Object2.Object_Valid[0|1],SensorOutput.Object3.Object_Valid[0|1],SensorOutput.Object4.Object_Valid[0|1],SensorOutput.Object5.Object_Valid[0|1]
  Bus Selector3 : BusSelector  OutputSignals=SensorOutput.Object1.CustomValues[],SensorOutput.Object2.CustomValues[],SensorOutput.Object3.CustomValues[],SensorOutput.Object4.CustomValues[],SensorOutput.Object5.CustomValues[]
  Bus Selector4 : BusSelector  OutputSignals=SensorOutput.Object1.CustomValues[],SensorOutput.Object2.CustomValues[],SensorOutput.Object3.CustomValues[],SensorOutput.Object4.CustomValues[],SensorOutput.Object5.CustomValues[]
  Bus Selector5 : BusSelector  OutputSignals=SensorOutput.Object1.CustomValues[],SensorOutput.Object2.CustomValues[],SensorOutput.Object3.CustomValues[],SensorOutput.Object4.CustomValues[],SensorOutput.Object5.CustomValues[]
  Mux : Mux  Inputs=15
  Mux1 : Mux  Inputs=15
  Vectorized_Custom_Values : Outport  VectorParamsAs1DForOutWhenUnconnected=off
  wires:
  Bus Creator/1 -> Vectorized_Custom_Values/1
  Bus Selector5/5 -> Mux1/15  "<CustomValues[]>"
  Bus Selector5/4 -> Mux1/14  "<CustomValues[]>"
  Bus Selector5/3 -> Mux1/13  "<CustomValues[]>"
  Bus Selector5/2 -> Mux1/12  "<CustomValues[]>"
  Bus Selector5/1 -> Mux1/11  "<CustomValues[]>"
  Bus Selector4/5 -> Mux1/10  "<CustomValues[]>"
  Bus Selector4/4 -> Mux1/9  "<CustomValues[]>"
  Bus Selector4/3 -> Mux1/8  "<CustomValues[]>"
  Bus Selector4/2 -> Mux1/7  "<CustomValues[]>"
  Bus Selector4/1 -> Mux1/6  "<CustomValues[]>"
  Bus Selector3/5 -> Mux1/5  "<CustomValues[]>"
  Bus Selector3/4 -> Mux1/4  "<CustomValues[]>"
  Bus Selector3/3 -> Mux1/3  "<CustomValues[]>"
  Bus Selector3/2 -> Mux1/2  "<CustomValues[]>"
  Bus Selector3/1 -> Mux1/1  "<CustomValues[]>"
  Bus Selector2/5 -> Mux/15  "<Object_Valid[0|1]>"
  Bus Selector2/4 -> Mux/14  "<Object_Valid[0|1]>"
  Bus Selector2/3 -> Mux/13  "<Object_Valid[0|1]>"
  Bus Selector2/2 -> Mux/12  "<Object_Valid[0|1]>"
  Bus Selector2/1 -> Mux/11  "<Object_Valid[0|1]>"
  Bus Selector1/5 -> Mux/10  "<Object_Valid[0|1]>"
  Bus Selector1/4 -> Mux/9  "<Object_Valid[0|1]>"
  Bus Selector1/3 -> Mux/8  "<Object_Valid[0|1]>"
  Bus Selector1/2 -> Mux/7  "<Object_Valid[0|1]>"
  Bus Selector1/1 -> Mux/6  "<Object_Valid[0|1]>"
  Mux1/1 -> Bus Creator/2  "CustomValues[]"
  Mux/1 -> Bus Creator/1  "Object_Valid[0|1]"
  SensorOutput3/1 -> Bus Selector2/1, Bus Selector5/1
  SensorOutput2/1 -> Bus Selector1/1, Bus Selector4/1
  Bus Selector/1 -> Mux/1  "<Object_Valid[0|1]>"
  Bus Selector/2 -> Mux/2  "<Object_Valid[0|1]>"
  Bus Selector/3 -> Mux/3  "<Object_Valid[0|1]>"
  Bus Selector/4 -> Mux/4  "<Object_Valid[0|1]>"
  Bus Selector/5 -> Mux/5  "<Object_Valid[0|1]>"
  SensorOutput1/1 -> Bus Selector3/1, Bus Selector/1

== system ASM_Traffic_MultiCore/Environment/Sensors/PlantModel/Object_Sensor_2D/ObjectData/Sensor7/Object_Custom_Values/Vectorize_Signals ==
  SensorOutput1 : Inport
  SensorOutput2 : Inport  Port=2
  SensorOutput3 : Inport  Port=3
  Bus Creator : BusCreator  Inputs=2
  Bus Selector : BusSelector  OutputSignals=SensorOutput.Object1.Object_Valid[0|1],SensorOutput.Object2.Object_Valid[0|1],SensorOutput.Object3.Object_Valid[0|1],SensorOutput.Object4.Object_Valid[0|1],SensorOutput.Object5.Object_Valid[0|1]
  Bus Selector1 : BusSelector  OutputSignals=SensorOutput.Object1.Object_Valid[0|1],SensorOutput.Object2.Object_Valid[0|1],SensorOutput.Object3.Object_Valid[0|1],SensorOutput.Object4.Object_Valid[0|1],SensorOutput.Object5.Object_Valid[0|1]
  Bus Selector2 : BusSelector  OutputSignals=SensorOutput.Object1.Object_Valid[0|1],SensorOutput.Object2.Object_Valid[0|1],SensorOutput.Object3.Object_Valid[0|1],SensorOutput.Object4.Object_Valid[0|1],SensorOutput.Object5.Object_Valid[0|1]
  Bus Selector3 : BusSelector  OutputSignals=SensorOutput.Object1.CustomValues[],SensorOutput.Object2.CustomValues[],SensorOutput.Object3.CustomValues[],SensorOutput.Object4.CustomValues[],SensorOutput.Object5.CustomValues[]
  Bus Selector4 : BusSelector  OutputSignals=SensorOutput.Object1.CustomValues[],SensorOutput.Object2.CustomValues[],SensorOutput.Object3.CustomValues[],SensorOutput.Object4.CustomValues[],SensorOutput.Object5.CustomValues[]
  Bus Selector5 : BusSelector  OutputSignals=SensorOutput.Object1.CustomValues[],SensorOutput.Object2.CustomValues[],SensorOutput.Object3.CustomValues[],SensorOutput.Object4.CustomValues[],SensorOutput.Object5.CustomValues[]
  Mux : Mux  Inputs=15
  Mux1 : Mux  Inputs=15
  Vectorized_Custom_Values : Outport  VectorParamsAs1DForOutWhenUnconnected=off
  wires:
  SensorOutput1/1 -> Bus Selector/1, Bus Selector3/1
  Bus Selector/5 -> Mux/5  "<Object_Valid[0|1]>"
  Bus Selector/4 -> Mux/4  "<Object_Valid[0|1]>"
  Bus Selector/3 -> Mux/3  "<Object_Valid[0|1]>"
  Bus Selector/2 -> Mux/2  "<Object_Valid[0|1]>"
  Bus Selector/1 -> Mux/1  "<Object_Valid[0|1]>"
  SensorOutput2/1 -> Bus Selector4/1, Bus Selector1/1
  SensorOutput3/1 -> Bus Selector5/1, Bus Selector2/1
  Mux/1 -> Bus Creator/1  "Object_Valid[0|1]"
  Mux1/1 -> Bus Creator/2  "CustomValues[]"
  Bus Selector1/1 -> Mux/6  "<Object_Valid[0|1]>"
  Bus Selector1/2 -> Mux/7  "<Object_Valid[0|1]>"
  Bus Selector1/3 -> Mux/8  "<Object_Valid[0|1]>"
  Bus Selector1/4 -> Mux/9  "<Object_Valid[0|1]>"
  Bus Selector1/5 -> Mux/10  "<Object_Valid[0|1]>"
  Bus Selector2/1 -> Mux/11  "<Object_Valid[0|1]>"
  Bus Selector2/2 -> Mux/12  "<Object_Valid[0|1]>"
  Bus Selector2/3 -> Mux/13  "<Object_Valid[0|1]>"
  Bus Selector2/4 -> Mux/14  "<Object_Valid[0|1]>"
  Bus Selector2/5 -> Mux/15  "<Object_Valid[0|1]>"
  Bus Selector3/1 -> Mux1/1  "<CustomValues[]>"
  Bus Selector3/2 -> Mux1/2  "<CustomValues[]>"
  Bus Selector3/3 -> Mux1/3  "<CustomValues[]>"
  Bus Selector3/4 -> Mux1/4  "<CustomValues[]>"
  Bus Selector3/5 -> Mux1/5  "<CustomValues[]>"
  Bus Selector4/1 -> Mux1/6  "<CustomValues[]>"
  Bus Selector4/2 -> Mux1/7  "<CustomValues[]>"
  Bus Selector4/3 -> Mux1/8  "<CustomValues[]>"
  Bus Selector4/4 -> Mux1/9  "<CustomValues[]>"
  Bus Selector4/5 -> Mux1/10  "<CustomValues[]>"
  Bus Selector5/1 -> Mux1/11  "<CustomValues[]>"
  Bus Selector5/2 -> Mux1/12  "<CustomValues[]>"
  Bus Selector5/3 -> Mux1/13  "<CustomValues[]>"
  Bus Selector5/4 -> Mux1/14  "<CustomValues[]>"
  Bus Selector5/5 -> Mux1/15  "<CustomValues[]>"
  Bus Creator/1 -> Vectorized_Custom_Values/1

== system ASM_Traffic_MultiCore/Environment/Sensors/PlantModel/Object_Sensor_3D/CustomPoints/Sensor1/CustomPointsOutput/HoldSignals ==
  ResetPulse[0|1] : Inport
  CustomPoints_Signals_In[] : Inport  Port=2
  Enable : EnablePort
  Bus Selector1 : BusSelector  OutputSignals=Flag_In_Scope[0|1],Flag_Is_Occluded[0|1],ID[],Dist_CoorSys_S[m],v_CoorSys_S[m|s],v_CoorSys_S[x;y;z][m|s],a_CoorSys_S[m|s2],a_CoorSys_S[x;y;z][m|s2],Pos_CoorSys_S[x;y;z][m],Pos_CoorSys_E[x;y;z][m],Angle_Hor_CoorSys_S[deg],Angle_Ver_CoorSys_S[deg],Data_1[],Data_2[],Data_3[],Data_4[],Data_5[],Object_ID[],Object_Type[]
  CUSTOM_POINTS_SIGNALS_RESET_1 : ASM_Traffic_lib/Sensors/Custom Points/CUSTOM_POINTS_SIGNALS_RESET  ASMProperties=struct('Name','CUSTOM_POINTS_SIGNALS_RESET','Version','2.0','Library','ASM_Traffic_lib')  ASMInstanceName=custom_points_signals_reset  ASMInstanceID=1
  CustomPoints_Signals_Out[] : Outport  VectorParamsAs1DForOutWhenUnconnected=off
  wires:
  Bus Selector1/19 -> CUSTOM_POINTS_SIGNALS_RESET_1/20  "<Object_Type[]>"
  Bus Selector1/18 -> CUSTOM_POINTS_SIGNALS_RESET_1/19  "<Object_ID[]>"
  Bus Selector1/17 -> CUSTOM_POINTS_SIGNALS_RESET_1/18  "<Data_5[]>"
  Bus Selector1/16 -> CUSTOM_POINTS_SIGNALS_RESET_1/17  "<Data_4[]>"
  Bus Selector1/15 -> CUSTOM_POINTS_SIGNALS_RESET_1/16  "<Data_3[]>"
  Bus Selector1/14 -> CUSTOM_POINTS_SIGNALS_RESET_1/15  "<Data_2[]>"
  Bus Selector1/13 -> CUSTOM_POINTS_SIGNALS_RESET_1/14  "<Data_1[]>"
  Bus Selector1/12 -> CUSTOM_POINTS_SIGNALS_RESET_1/13  "<Angle_Ver_CoorSys_S[deg]>"
  Bus Selector1/11 -> CUSTOM_POINTS_SIGNALS_RESET_1/12  "<Angle_Hor_CoorSys_S[deg]>"
  Bus Selector1/10 -> CUSTOM_POINTS_SIGNALS_RESET_1/11  "<Pos_CoorSys_E[x;y;z][m]>"
  Bus Selector1/9 -> CUSTOM_POINTS_SIGNALS_RESET_1/10  "<Pos_CoorSys_S[x;y;z][m]>"
  Bus Selector1/8 -> CUSTOM_POINTS_SIGNALS_RESET_1/9  "<a_CoorSys_S[x;y;z][m|s2]>"
  Bus Selector1/7 -> CUSTOM_POINTS_SIGNALS_RESET_1/8  "<a_CoorSys_S[m|s2]>"
  Bus Selector1/6 -> CUSTOM_POINTS_SIGNALS_RESET_1/7  "<v_CoorSys_S[x;y;z][m|s]>"
  Bus Selector1/5 -> CUSTOM_POINTS_SIGNALS_RESET_1/6  "<v_CoorSys_S[m|s]>"
  Bus Selector1/4 -> CUSTOM_POINTS_SIGNALS_RESET_1/5  "<Dist_CoorSys_S[m]>"
  Bus Selector1/3 -> CUSTOM_POINTS_SIGNALS_RESET_1/4  "<ID[]>"
  Bus Selector1/2 -> CUSTOM_POINTS_SIGNALS_RESET_1/3  "<Flag_Is_Occluded[0|1]>"
  Bus Selector1/1 -> CUSTOM_POINTS_SIGNALS_RESET_1/2  "<Flag_In_Scope[0|1]>"
  CUSTOM_POINTS_SIGNALS_RESET_1/1 -> CustomPoints_Signals_Out[]/1
  ResetPulse[0|1]/1 -> CUSTOM_POINTS_SIGNALS_RESET_1/1
  CustomPoints_Signals_In[]/1 -> Bus Selector1/1
